simulink model "exp1"  (R2018b)
settings: Solver=ode45  StartTime=0.0  StopTime=30.0  RelTol=1e-3
settings Model: Creator=lenovo  LastModifiedBy=lenovo

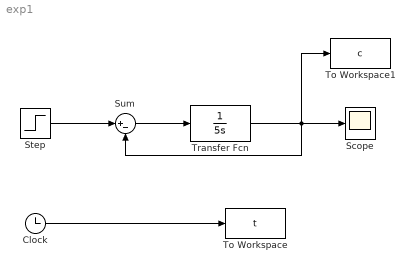
== system exp1 ==
  Clock : Clock
  Scope : Scope
  Step : Step  SampleTime=0
  Sum : Sum  Inputs=|+-
  To Workspace : ToWorkspace  VariableName=t  SampleTime=-1
  To Workspace1 : ToWorkspace  VariableName=c  SampleTime=-1
  Transfer Fcn : TransferFcn  Denominator=[5 0]
  wires:
  Step/1 -> Sum/1
  Sum/1 -> Transfer Fcn/1
  Transfer Fcn/1 -> To Workspace1/1, Sum/2, Scope/1
  Clock/1 -> To Workspace/1
